simulink model "quadcopter_ex03_wind_conditions"  (R2025b)
settings: Solver=VariableStepAuto  StartTime=0.0  StopTime=200  MaxStep=0.01  RelTol=1e-3
Description:
  | Copyright 2022-2025 The MathWorks, Inc.
settings Model: Creator=smiller  LastModifiedBy=smiller
settings OptimizationCC: ReuseModelBlockBuffer=off
settings DebuggingCC: UnconnectedInputMsg=warning  UnconnectedOutputMsg=warning  UnconnectedLineMsg=warning
settings ModelReferenceCC: EnableRefExpFcnMdlSchedulingChecks=on
settings RTWCC: GPUComputeCapability=3.5  DLArmComputeVersion=19.05

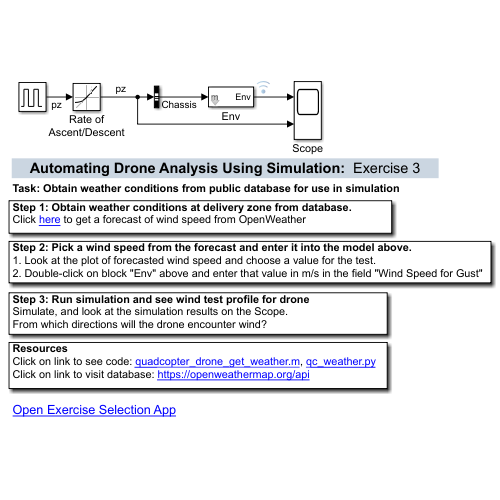
[thumbnail: Simulink's stored preview of the top-level diagram]
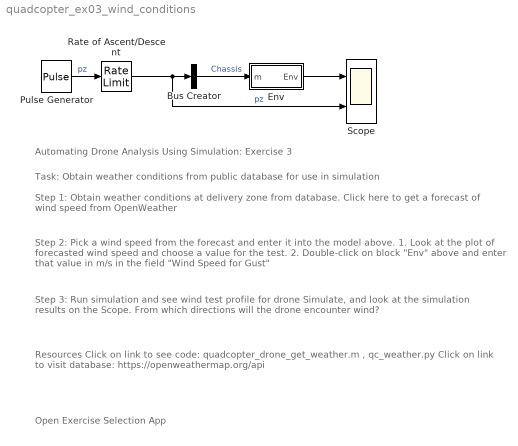
== system quadcopter_ex03_wind_conditions ==
  note: Automating Drone Analysis Using Simulation: Exercise 3
  note: Step 1: Obtain weather conditions at delivery zone from database.
      | Click here to get a forecast of wind speed from OpenWeather
  note: Task: Obtain weather conditions from public database for use in simulation
  note: Step 2: Pick a wind speed from the forecast and enter it into the model above.
      | 1. Look at the plot of forecasted wind speed and choose a value for the test.
      | 2. Double-click on block "Env" above and enter that value in m/s in the field "Wind Speed for Gust"
  note: Step 3: Run simulation and see wind test profile for drone
      | Simulate, and look at the simulation results on the Scope.
      | From which directions will the drone encounter wind?
  note: Resources
      | Click on link to see code: quadcopter_drone_get_weather.m , qc_weather.py
      | Click on link to visit database: https://openweathermap.org/api
  note: Open Exercise Selection App
  Bus Creator : BusCreator  Inputs=1
  Env : Subsystem  mask{wind_speed_mag=5, height_max_wind=6, height_min_wind=2}
      mask prompts: wind_speed_mag "Wind Speed for Gust (m/s)"; height_max_wind "Lowest Height for Max Wind (m)"; height_min_wind "Maximum Height for Zero Wind (m)"
  Pulse Generator : DiscretePulseGenerator  PulseType=Time based  Amplitude=6  Period=100  PulseWidth=70  PhaseDelay=10
  Rate of Ascent/Descent : RateLimiter  RisingSlewLimit=6/20  FallingSlewLimit=-6/20  SampleTimeMode=inherited
  Scope : Scope  NumInputPorts=2
      settings: Title=Wind Speed (global x, y, z)  ActiveDisplayYMinimum=-1.25  ActiveDisplayYMaximum=11.25  YLabel=m/s
  wires:
  Rate of Ascent/Descent/1 -> Scope/2, Bus Creator/1  "pz"
  Bus Creator/1 -> Env/1(m)  "Chassis"
  Env/1(Env) -> Scope/1
  Pulse Generator/1 -> Rate of Ascent/Descent/1  "pz"

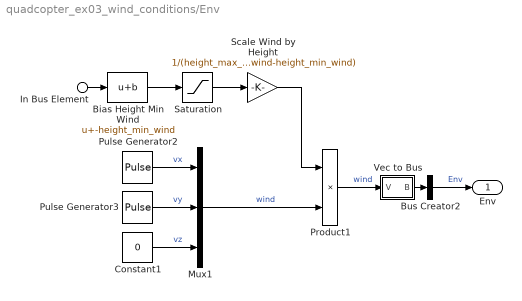
== system quadcopter_ex03_wind_conditions/Env ==
  In Bus Element : Inport  PortName=m  Element=pz
  Bias Height Min Wind : Bias  Bias=-height_min_wind  SaturateOnIntegerOverflow=off
  Bus Creator2 : BusCreator  Inputs=1
  Constant1 : Constant  Value=0
  Mux1 : Mux  Inputs=3
  Product1 : Product
  Pulse Generator2 : DiscretePulseGenerator  PulseType=Time based  Amplitude=wind_speed_mag  Period=10  PulseWidth=25  PhaseDelay=5
  Pulse Generator3 : DiscretePulseGenerator  PulseType=Time based  Amplitude=wind_speed_mag  Period=10  PulseWidth=25  PhaseDelay=9
  Saturation : Saturate  UpperLimit=height_max_wind-height_min_wind  LowerLimit=0  ZeroCross=off
  "Scale Wind by Height " : Gain  Gain=1/(height_max_wind-height_min_wind)
  Vec to Bus : Subsystem
  Env : Outport
  wires:
  In Bus Element/1 -> Bias Height Min Wind/1
  Bias Height Min Wind/1 -> Saturation/1
  Saturation/1 -> "Scale Wind by Height "/1
  "Scale Wind by Height "/1 -> Product1/1
  Constant1/1 -> Mux1/3  "vz"
  Pulse Generator3/1 -> Mux1/2  "vy"
  Pulse Generator2/1 -> Mux1/1  "vx"
  Mux1/1 -> Product1/2  "wind"
  Product1/1 -> Vec to Bus/1(V)  "wind"
  Vec to Bus/1(B) -> Bus Creator2/1
  Bus Creator2/1 -> Env/1  "Env"

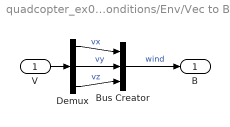
== system quadcopter_ex03_wind_conditions/Env/Vec to Bus ==
  V : Inport
  Bus Creator : BusCreator  Inputs=3
  Demux : Demux  Outputs=3
  B : Outport
  wires:
  Demux/3 -> Bus Creator/3  "vz"
  V/1 -> Demux/1
  Demux/1 -> Bus Creator/1  "vx"
  Demux/2 -> Bus Creator/2  "vy"
  Bus Creator/1 -> B/1  "wind"
